simulink model "TempControl_OpenLoop_sakai_2024"  (R2024b)
settings: Solver=FixedStepDiscrete  StartTime=0.0  StopTime=600  FixedStep=10e-3  RelTol=1e-3  EnableMultiTasking=on
values from neighbouring files (symbols this model uses):
  Kmeas = Vref/S_LM35    (= 330)    [prep_lab_1.m]
libraries: mbedblockslib x2
settings Model: ExtModeTrigDuration=10  Creator=Lukas  LastModifiedBy=Lukas
settings OptimizationCC: EnhancedBackFolding=on  PassReuseOutputArgsAs=Individual arguments  ZeroExternalMemoryAtStartup=off  ZeroInternalMemoryAtStartup=off  MaxStackSize=64  OptimizeBlockOrder=speed  DifferentSizesBufferReuse=on  OptimizationCustomize=off  EfficientTunableParamExpr=on
settings DebuggingCC: ParameterTunabilityLossMsg=error
settings HardwareCC: ProdBitPerPointer=32  ProdBitPerSizeT=32  ProdBitPerPtrDiffT=32  ProdLargestAtomicInteger=Long  ProdLargestAtomicFloat=Double  ProdWordSize=32  ProdLongLongMode=on  ProdHWDeviceType=ARM Compatible->ARM Cortex  UseEmbeddedCoderFeatures=off
settings SFSimCC: MATLABDynamicMemAlloc=off
settings RTWCC: Description=Embedded Coder  SystemTargetFile=ert.tlc  HardwareBoard=STM32 Nucleo F401RE  TemplateMakefile=ert_default_tmf  GPUComputeCapability=3.5
settings CodeAppCC: ForceParamTrailComments=on  IgnoreCustomStorageClasses=off  OperatorAnnotations=on  SimulinkDataObjDesc=on  SFDataObjDesc=on  InsertBlockDesc=on
settings ERTTargetCC: CodeReplacementLibrary=ARM Cortex-M  SupportNonInlinedSFcns=on  ExtModeTransport=3  ExtModeStaticAlloc=on  ExtModeStaticAllocSize=2000  ExtModeMexFile=ext_xcp  ExtModeIntrfLevel=Level2 - Open  InlinedParameterPlacement=Hierarchical  DynamicArrayContainerType=coder::array
settings ConfigComp: CovMetricSettings=de  CovBoundaryAbsTol=1.0e-5

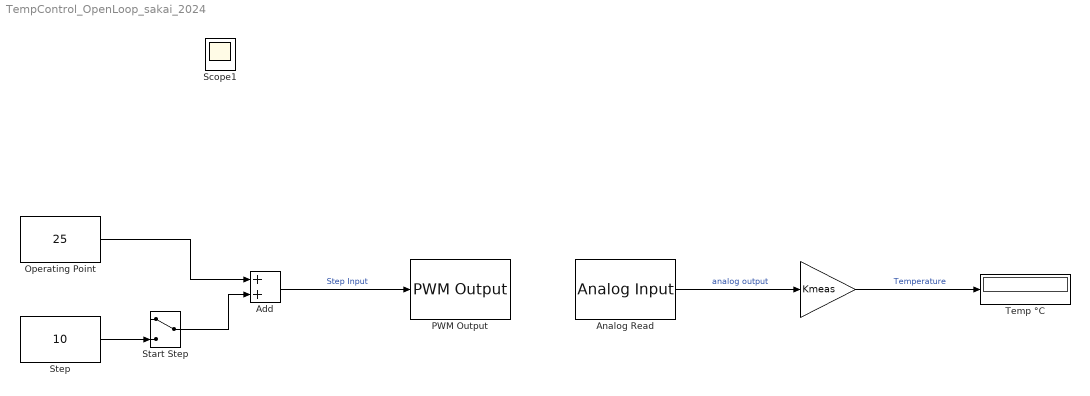
== system TempControl_OpenLoop_sakai_2024 ==
  " " : Gain  Gain=Kmeas
  Add : Sum
  Analog Read : mbedblockslib/Analog Input  Pin=A0  ReadResultsOnly=off  ConversionTriggerSource=Software  ExternalTriggerType=uint32( 0 )  OutputDataType=double  EnableConversionCompleteNotify=off  EnableOuputStatus=off  SampleTime=10e-3
      settings: LibrarySourceBlock=stmnucleorootlib/Common/Analog Input
  Operating Point : Constant  Value=25  SampleTime=10e-3
  PWM Output : mbedblockslib/PWM Output  Pin=D2  EnableInputFrequency=off  InitialFrequency=10000  InitialDutyCycle=20  NotificationType=None
      settings: LibrarySourceBlock=stmnucleorootlib/Common/PWM Output
  Start Step : ManualSwitch
  Step : Constant  Value=10  SampleTime=10e-3
  Temp °C : Display
  Scope1 : Scope
  wires:
  Operating Point/1 -> Add/1
  Add/1 -> PWM Output/1  "Step Input"
  Step/1 -> Start Step/2
  Start Step/1 -> Add/2
  Analog Read/1 -> " "/1  "analog output"
  " "/1 -> Temp °C/1  "Temperature"
